simulink model "ConfiguredHevMmVirtualVehicle"  (R2025b)
settings: configuration reference "VehicleVariable" (kept outside this file)
StartFcn:
  | %tic
StopFcn:
  | %toc
model workspace (MAT data in the model file):
  ExtDrvCmdsSwitch : Simulink.Parameter (value not decoded)
  ExtDrvRefSwitch : Simulink.Parameter (value not decoded)
  ExtEnvSwitch : Simulink.Parameter (value not decoded)
  ExtGndSwitch : Simulink.Parameter (value not decoded)
symbols that are objects in the model workspace (value not decoded): ExtDrvCmdsSwitch, ExtDrvRefSwitch, ExtEnvSwitch, ExtGndSwitch
undefined symbols (not defined in the file or in its folder): AmbTemp, BaroPress, CurvGradRef, CurvRef, DCM, DriverAeroRes, DriverDrivelineRes, DriverInitialGear, DriverPreviewDist, DriverRollRes, DriverShiftTime, DriverTimeConst, DriverTractiveForce, EnvAbsPrs, EnvAirTemp, EnvGrvty, EnvNomFrictionScaling, EnvNominalGrade, EnvScnFrictionMap, EnvScnFrictionMapXBpts, EnvScnFrictionMapYBpts, EnvScnHeightMap, EnvScnHeightMapXBpts, EnvScnHeightMapYBpts, EnvWindVelX, EnvWindVelY, EnvWindVelZ, Gnd, Grade, HazzardCmd, HighBeamCmd, lambda_mux, LeftSignalCmd, LngRef, LowBeamCmd, LtrRef, PhiRef, PlntVehDstCGFrntAxl, PlntVehDstCGRearAxl, PlntVehInitLatPos, PlntVehInitLongPos, PlntVehInitPitchAng, PlntVehInitRollAng, PlntVehInitVertPos, PlntVehInitYawAng, PlntVehMass, PlntVehTrckWdth, PlntVehYawMomentInertia, PlntWhlLdRadiusFrnt, PlntWhlLdRadiusRear, RightSignalCmd, ScnCRRadius, Sim3dSensor, Wind, XRef, YRef, Z
libraries: simulink x28, autolibutils x8, autolibsharedcommon x7, vehdynlibscenariocommon x7, vehdynlibviscommon x4, vehdynlibdriver x2, sim3dgroundtruthsensorlib x2, sim3dlib x2, autolibshared x2, sim3dautolib x2, sl3dlib x1, sharedtransform x1
(part 5 of 6)

== system ConfiguredHevMmVirtualVehicle/Driver Commands/Driver Commands/Longitudinal Driver/Hill Hold & Stop ==
  LngRef : Inport
  <EnblDecelCmd> : Inport  Port=2
  <DecelOvrCmd> : Inport  Port=3
  <DecelHld> : Inport  Port=4
  <DecelZero> : Inport  Port=5
  Env : Inport  Port=6
  VehFdbk : Inport  Port=7
  Bus Selector : BusSelector  OutputSignals=Engine.EngSpdOut,Body.BdyFrm.Cg.Vel.xdot,Battery.BattInfo.BattSoc
  Bus Selector1 : BusSelector  OutputSignals=Body.BdyFrm.Cg.Vel.xdot
  Bus Selector2 : BusSelector  OutputSignals=Grade
  Hill Hold : Subsystem
  Logical Operator4 : Logic  Operator=OR  AllPortsSameDT=off  OutDataTypeStr=boolean
  Max : MinMax  Function=max  Inputs=2  ZeroCross=off
  Stop Detection : Subsystem
  Switch : Switch  Criteria=u2 > Threshold  SaturateOnIntegerOverflow=off  InputSameDT=off
  Switch1 : Switch  Criteria=u2 > Threshold  SaturateOnIntegerOverflow=off  InputSameDT=off
  VehFdbk1 : InportShadow  Port=7
  EnblDecelOvr : Outport
  DecelOvrCmd : Outport  Port=2
  DecelHld : Outport  Port=3
  DecelZero : Outport  Port=4
  VelFdbk : Outport  Port=5
  Grade : Outport  Port=6
  wires:
  Hill Hold/1(DecelOvr) -> Logical Operator4/1
  Hill Hold/2(EnblDecelOvr) -> Max/1
  Bus Selector/3 -> Hill Hold/3(<BattSoc>)  "<BattSoc>"
  Bus Selector/2 -> Hill Hold/2(<xdot>)  "<xdot>"
  Bus Selector/1 -> Hill Hold/1(<EngSpdOut>)  "<EngSpdOut>"
  Stop Detection/1(DecelOvrCmd) -> Max/2
  Stop Detection/2(EnblDecelOvr) -> Logical Operator4/2
  Logical Operator4/1 -> Switch/3
  Switch1/1 -> DecelOvrCmd/1
  Switch/1 -> EnblDecelOvr/1
  <EnblDecelCmd>/1 -> Switch1/2, Switch/1, Switch/2
  Max/1 -> Switch1/3
  Bus Selector1/1 -> VelFdbk/1, Stop Detection/2(<xdot>)  "<xdot>"
  LngRef/1 -> Hill Hold/4(LngRef), Stop Detection/1(LngRef)
  VehFdbk/1 -> Bus Selector/1
  <DecelOvrCmd>/1 -> Switch1/1
  Env/1 -> Bus Selector2/1
  Bus Selector2/1 -> Hill Hold/5(<Grade>), Grade/1  "<Grade>"
  VehFdbk1/1 -> Bus Selector1/1
  <DecelZero>/1 -> DecelZero/1
  <DecelHld>/1 -> DecelHld/1

== system ConfiguredHevMmVirtualVehicle/Driver Commands/Driver Commands/Longitudinal Driver/Longitudinal Driver ==
  VelRef : Inport  Unit=m/s
  EnblAccelOvr : Inport  Port=2
  AccelOvrCmd : Inport  Port=3
  AccelHld : Inport  Port=4
  AccelZero : Inport  Port=5
  EnblDecelOvr : Inport  Port=6
  DecelOvrCmd : Inport  Port=7
  DecelHld : Inport  Port=8
  DecelZero : Inport  Port=9
  VelFdbk : Inport  Port=10  Unit=m/s
  Grade : Inport  Port=11
  ExtGearGround : Ground
  External Action Routing : Subsystem
  Longitudinal Driver : autolibsharedcommon/Longitudinal Driver  cntrlType=PI  shftType=Reverse, Neutral, Drive  vnom=vnom  Kp=Kp  Ki=Ki  Kaw=Kaw  Kff=Kff  Kg=Kg  tauerr=tauerr  tShift=tShift  tRev=tRev  tPark=tPark  pdlVec=pdlVec  upShftTbl=upShftTbl  dwnShftTbl=dwnShftTbl  GearInit=GearInit  tClutch=tClutch  VehVelVec=VehVelVec  KffVec=KffVec  KiVec=KiVec  KpVec=KpVec  KgVec=KgVec  m=m  Kpt=Kpt  Lvv=L  g=g  UpGearVec=UpGearVec  DownGearVec=DownGearVec  aMode=6  errUnit=m/s  aR=aR  bR=bR  cR=cR  tauPt=tauPt
      settings: LibrarySourceBlock=autolibshared/Longitudinal Driver/Longitudinal Driver
  Info : Outport  InitialOutput=0  VectorParamsAs1DForOutWhenUnconnected=off
  AccelCmd : Outport  Port=2  VectorParamsAs1DForOutWhenUnconnected=off
  DecelCmd : Outport  Port=3  VectorParamsAs1DForOutWhenUnconnected=off
  GearCmd : Outport  Port=4
  wires:
  DecelZero/1 -> External Action Routing/8(DecelZero)
  DecelHld/1 -> External Action Routing/7(DecelHld)
  DecelOvrCmd/1 -> External Action Routing/6(DecelOvrCmd)
  EnblDecelOvr/1 -> External Action Routing/5(EnblDecelOvr)
  AccelZero/1 -> External Action Routing/4(AccelZero)
  AccelHld/1 -> External Action Routing/3(AccelHld)
  AccelOvrCmd/1 -> External Action Routing/2(AccelOvrCmd)
  EnblAccelOvr/1 -> External Action Routing/1(EnblAccelOvr)
  Longitudinal Driver/4 -> GearCmd/1
  ExtGearGround/1 -> Longitudinal Driver/4
  External Action Routing/1(ExtActions) -> Longitudinal Driver/5
  Grade/1 -> Longitudinal Driver/3
  Longitudinal Driver/3 -> DecelCmd/1
  Longitudinal Driver/2 -> AccelCmd/1
  Longitudinal Driver/1 -> Info/1
  VelFdbk/1 -> Longitudinal Driver/2
  VelRef/1 -> Longitudinal Driver/1

== system ConfiguredHevMmVirtualVehicle/Driver Commands/Driver Commands/Predictive Driver/Hill Hold & Stop ==
  LngRef : Inport
  <EnblDecelCmd> : Inport  Port=2
  <DecelOvrCmd> : Inport  Port=3
  <DecelHld> : Inport  Port=4
  <DecelZero> : Inport  Port=5
  Env : Inport  Port=6
  VehFdbk : Inport  Port=7
  Bus Selector : BusSelector  OutputSignals=Engine.EngSpdOut,Body.BdyFrm.Cg.Vel.xdot,Battery.BattInfo.BattSoc
  Bus Selector1 : BusSelector  OutputSignals=Body.BdyFrm.Cg.Vel.xdot
  Bus Selector2 : BusSelector  OutputSignals=Grade
  Hill Hold : Subsystem
  Logical Operator4 : Logic  Operator=OR  AllPortsSameDT=off  OutDataTypeStr=boolean
  Max : MinMax  Function=max  Inputs=2
  Stop Detection : Subsystem
  Switch : Switch  Criteria=u2 > Threshold  SaturateOnIntegerOverflow=off  InputSameDT=off
  Switch1 : Switch  Criteria=u2 > Threshold  SaturateOnIntegerOverflow=off  InputSameDT=off
  VehFdbk1 : InportShadow  Port=7
  EnblDecelOvr : Outport
  DecelOvrCmd : Outport  Port=2
  DecelHld : Outport  Port=3
  DecelZero : Outport  Port=4
  Grade : Outport  Port=5
  VelFdbk : Outport  Port=6
  wires:
  Hill Hold/1(DecelOvr) -> Logical Operator4/1
  Hill Hold/2(EnblDecelOvr) -> Max/1
  Bus Selector/3 -> Hill Hold/3(<BattSoc>)  "<BattSoc>"
  Bus Selector/2 -> Hill Hold/2(<xdot>)  "<xdot>"
  Bus Selector/1 -> Hill Hold/1(<EngSpdOut>)  "<EngSpdOut>"
  Stop Detection/1(DecelOvrCmd) -> Max/2
  Stop Detection/2(EnblDecelOvr) -> Logical Operator4/2
  Logical Operator4/1 -> Switch/3
  Switch1/1 -> DecelOvrCmd/1
  Switch/1 -> EnblDecelOvr/1
  <EnblDecelCmd>/1 -> Switch1/2, Switch/1, Switch/2
  Max/1 -> Switch1/3
  Bus Selector1/1 -> VelFdbk/1, Stop Detection/2(<xdot>)  "<xdot>"
  LngRef/1 -> Hill Hold/4(LngRef), Stop Detection/1(LngRef)
  VehFdbk/1 -> Bus Selector/1
  <DecelOvrCmd>/1 -> Switch1/1
  Env/1 -> Bus Selector2/1
  Bus Selector2/1 -> Hill Hold/5(<Grade>), Grade/1  "<Grade>"
  VehFdbk1/1 -> Bus Selector1/1
  <DecelZero>/1 -> DecelZero/1
  <DecelHld>/1 -> DecelHld/1

== system ConfiguredHevMmVirtualVehicle/Driver Commands/Driver Commands/Predictive Stanley Driver/Hill Hold & Stop ==
  LngRef : Inport
  <EnblDecelCmd> : Inport  Port=2
  <DecelOvrCmd> : Inport  Port=3
  <DecelHld> : Inport  Port=4
  <DecelZero> : Inport  Port=5
  <CurvRef> : Inport  Port=6
  Env : Inport  Port=7
  VehFdbk : Inport  Port=8
  Bus Selector : BusSelector  OutputSignals=Engine.EngSpdOut,Body.BdyFrm.Cg.Vel.xdot,Battery.BattInfo.BattSoc
  Bus Selector1 : BusSelector  OutputSignals=Body.BdyFrm.Cg.Vel.xdot
  Bus Selector2 : BusSelector  OutputSignals=Grade
  Hill Hold : Subsystem
  Logical Operator4 : Logic  Operator=OR  AllPortsSameDT=off  OutDataTypeStr=boolean
  Max : MinMax  Function=max  Inputs=2
  Stop Detection : Subsystem
  Switch : Switch  Criteria=u2 > Threshold  SaturateOnIntegerOverflow=off  InputSameDT=off
  Switch1 : Switch  Criteria=u2 > Threshold  SaturateOnIntegerOverflow=off  InputSameDT=off
  VehFdbk1 : InportShadow  Port=8
  EnblDecelOvr : Outport
  DecelOvrCmd : Outport  Port=2
  DecelHld : Outport  Port=3
  DecelZero : Outport  Port=4
  Grade : Outport  Port=5
  CurvRef : Outport  Port=6
  VelFdbk : Outport  Port=7
  wires:
  Hill Hold/1(DecelOvr) -> Logical Operator4/1
  Hill Hold/2(EnblDecelOvr) -> Max/1
  Bus Selector/3 -> Hill Hold/3(<BattSoc>)  "<BattSoc>"
  Bus Selector/2 -> Hill Hold/2(<xdot>)  "<xdot>"
  Bus Selector/1 -> Hill Hold/1(<EngSpdOut>)  "<EngSpdOut>"
  Stop Detection/1(DecelOvrCmd) -> Max/2
  Stop Detection/2(EnblDecelOvr) -> Logical Operator4/2
  Logical Operator4/1 -> Switch/3
  Switch1/1 -> DecelOvrCmd/1
  Switch/1 -> EnblDecelOvr/1
  <EnblDecelCmd>/1 -> Switch1/2, Switch/1, Switch/2
  Max/1 -> Switch1/3
  Bus Selector1/1 -> VelFdbk/1, Stop Detection/2(<xdot>)  "<xdot>"
  LngRef/1 -> Hill Hold/4(LngRef), Stop Detection/1(LngRef)
  <CurvRef>/1 -> CurvRef/1
  VehFdbk/1 -> Bus Selector/1
  <DecelOvrCmd>/1 -> Switch1/1
  Env/1 -> Bus Selector2/1
  Bus Selector2/1 -> Hill Hold/5(<Grade>), Grade/1  "<Grade>"
  VehFdbk1/1 -> Bus Selector1/1
  <DecelZero>/1 -> DecelZero/1
  <DecelHld>/1 -> DecelHld/1

== system ConfiguredHevMmVirtualVehicle/Environment/Ground Feedback/3D Engine/3D Engine Source ==
  WheelFdbk : Inport
  Multiple Points : Subsystem  VariantControl=terrType==2
  Single Point : Subsystem  VariantControl=terrType ==1
  z : Outport
  DCM : Outport  Port=2

== system ConfiguredHevMmVirtualVehicle/Environment/Ground Feedback/Height Map/2D Lookup Tbl for Elevation, Z ==
  XWhl : Inport  Partition=on  PartitionDimension=1  PartitionWidth=1  PartitionOffset=0
  YWhl : Inport  Port=2  Partition=on  PartitionDimension=1  PartitionWidth=1  PartitionOffset=0
  2-D Lookup Table : Lookup_n-D  BreakpointsForDimension1=EnvScnHeightMapXBpts  BreakpointsForDimension2=EnvScnHeightMapYBpts  BeginIndexSearchUsingPreviousIndexResult=on  Table=EnvScnHeightMap  ExtrapMethod=Clip  InternalRulePriority=Speed  RndMeth=Simplest
      settings: InputPortMap=u0,u1
  Add : Sum
  Add1 : Sum
  Constant : Constant  Value=0
  Constant1 : Constant  Value=0
  For Each : ForEach  DisableCoverage=on
  Unary Minus : UnaryMinus
  Z : Outport  ConcatenationDimension=1
  wires:
  2-D Lookup Table/1 -> Z/1
  YWhl/1 -> Unary Minus/1
  XWhl/1 -> Add1/2
  Unary Minus/1 -> Add/1
  Add/1 -> 2-D Lookup Table/2
  Constant/1 -> Add/2
  Constant1/1 -> Add1/1
  Add1/1 -> 2-D Lookup Table/1

== system ConfiguredHevMmVirtualVehicle/Environment/Ground Feedback/Height Map/Wheel Coordinates ==
  FrntAxlLftX : Inport
  FrntAxlRghtX : Inport  Port=2
  RearAxlLftX : Inport  Port=3
  RearAxlRghtX : Inport  Port=4
  FrntAxlLftY : Inport  Port=5
  FrntAxlRghtY : Inport  Port=6
  RearAxlLftY : Inport  Port=7
  RearAxlRghtY : Inport  Port=8
  Matrix Concatenate : Concatenate  NumInputs=4  Mode=Multidimensional array
  Matrix Concatenate1 : Concatenate  NumInputs=4  Mode=Multidimensional array
  XWhl : Outport
  YWhl : Outport  Port=2
  wires:
  Matrix Concatenate1/1 -> YWhl/1
  FrntAxlLftX/1 -> Matrix Concatenate/1
  FrntAxlLftY/1 -> Matrix Concatenate1/1
  FrntAxlRghtY/1 -> Matrix Concatenate1/2
  FrntAxlRghtX/1 -> Matrix Concatenate/2
  RearAxlLftY/1 -> Matrix Concatenate1/3
  RearAxlLftX/1 -> Matrix Concatenate/3
  RearAxlRghtY/1 -> Matrix Concatenate1/4
  Matrix Concatenate/1 -> XWhl/1
  RearAxlRghtX/1 -> Matrix Concatenate/4

== system ConfiguredHevMmVirtualVehicle/Environment/Ground Feedback/Ideal Inclined Plane/Ideal Inclined Plane ==
  X : Inport
  Y : Inport  Port=2
  phi : Inport  Port=3
  theta : Inport  Port=4
  Constant : Constant  Value=Z_est
  Enabled : Subsystem  Variant=on
  Signal Specification1 : SignalSpecification  Unit=rad
  Signal Specification3 : SignalSpecification  Unit=rad
  Signal Specification4 : SignalSpecification  Unit=m
  Signal Specification5 : SignalSpecification  Unit=m
  Signal Specification6 : SignalSpecification  Unit=m
  Z Plane : MATLAB Function  InitFcn=|  TreatAsAtomicUnit=on
      | if builtin('license','test','Vehicle_Dynamics_Blockset')
      |    [~]=builtin('license','checkout','Vehicle_Dynamics_Blockset');
      | else
      |    error(message('autoblks_shared:autosharederrAutoIcon:invalidLicense'));
      | end
      mask init:
      | if builtin('license','test','Vehicle_Dynamics_Blockset')
      |     [~]=builtin('license','checkout','Vehicle_Dynamics_Blockset');
      | else
      |     error(message('autoblks_shared:autosharederrAutoIcon:invalidLicense'));
      | end
  Z : Outport
  DCM : Outport  Port=2
  wires:
  Z Plane/2(DCM) -> DCM/1
  Signal Specification1/1 -> Z Plane/5(theta), Enabled/3(theta)
  phi/1 -> Signal Specification3/1
  theta/1 -> Signal Specification1/1
  Signal Specification3/1 -> Z Plane/4(phi), Enabled/2(phi)
  Y/1 -> Signal Specification6/1
  Z Plane/1(Z) -> Signal Specification4/1
  X/1 -> Signal Specification5/1
  Signal Specification4/1 -> Z/1
  Signal Specification5/1 -> Z Plane/1(X)
  Signal Specification6/1 -> Z Plane/2(Y)
  Constant/1 -> Enabled/1(Z), Z Plane/3(Zoffset)

== system ConfiguredHevMmVirtualVehicle/Environment/Ground Feedback/Ideal Inclined Plane/Wheel Coordinates ==
  FrntAxlLftX : Inport
  FrntAxlRghtX : Inport  Port=2
  RearAxlLftX : Inport  Port=3
  RearAxlRghtX : Inport  Port=4
  FrntAxlLftY : Inport  Port=5
  FrntAxlRghtY : Inport  Port=6
  RearAxlLftY : Inport  Port=7
  RearAxlRghtY : Inport  Port=8
  Matrix Concatenate : Concatenate  NumInputs=4  Mode=Multidimensional array
  Matrix Concatenate1 : Concatenate  NumInputs=4  Mode=Multidimensional array
  XWhl : Outport
  YWhl : Outport  Port=2
  wires:
  RearAxlRghtX/1 -> Matrix Concatenate/4
  Matrix Concatenate/1 -> XWhl/1
  RearAxlRghtY/1 -> Matrix Concatenate1/4
  RearAxlLftX/1 -> Matrix Concatenate/3
  RearAxlLftY/1 -> Matrix Concatenate1/3
  FrntAxlRghtX/1 -> Matrix Concatenate/2
  FrntAxlRghtY/1 -> Matrix Concatenate1/2
  FrntAxlLftY/1 -> Matrix Concatenate1/1
  FrntAxlLftX/1 -> Matrix Concatenate/1
  Matrix Concatenate1/1 -> YWhl/1

== system ConfiguredHevMmVirtualVehicle/Environment/Subsystem/Estimated Grade/Variant Subsystem ==
  note: 1) Add Subsystem or Model blocks as valid variant choices.
      | 2) You cannot connect blocks at this level. At simulation, connectivity is automatically
      | determined, based on the active variant and port name matching.
  Gnd : Inport
  Three-Axle : Subsystem  VariantControl=ThreeAxle
  Two-Axle : Subsystem  VariantControl=TwoAxle
  F : Outport
  R : Outport  Port=2

== system ConfiguredHevMmVirtualVehicle/Environment/Subsystem/Variant Subsystem/Three-Axle ==
  InGnd : Inport
  Bus Selector1 : BusSelector  OutputSignals=z.G_FL_z,z.G_FR_z,z.G_ML_z,z.G_MR_z,z.G_RL_z,z.G_RR_z,DCM,mu.mu_FL,mu.mu_FR,mu.mu_ML,mu.mu_MR,mu.mu_RL,mu.mu_RR
  Mux : Mux  Inputs=6
  Mux1 : Mux  Inputs=6
  z : Outport
  <DCM> : Outport  Port=2
  lambda_mux : Outport  Port=3
  wires:
  Bus Selector1/12 -> Mux1/5  "<mu_RL>"
  Bus Selector1/7 -> <DCM>/1  "<DCM>"
  InGnd/1 -> Bus Selector1/1
  Bus Selector1/10 -> Mux1/3  "<mu_ML>"
  Bus Selector1/4 -> Mux/4  "<G_MR_z>"
  Bus Selector1/5 -> Mux/5  "<G_RL_z>"
  Bus Selector1/3 -> Mux/3  "<G_ML_z>"
  Bus Selector1/2 -> Mux/2  "<G_FR_z>"
  Bus Selector1/9 -> Mux1/2  "<mu_FR>"
  Bus Selector1/6 -> Mux/6  "<G_RR_z>"
  Mux/1 -> z/1
  Bus Selector1/11 -> Mux1/4  "<mu_MR>"
  Bus Selector1/1 -> Mux/1  "<G_FL_z>"
  Bus Selector1/13 -> Mux1/6  "<mu_RR>"
  Mux1/1 -> lambda_mux/1
  Bus Selector1/8 -> Mux1/1  "<mu_FL>"

== system ConfiguredHevMmVirtualVehicle/Environment/Subsystem/Variant Subsystem/Two-Axle ==
  InGnd : Inport
  Bus Selector1 : BusSelector  OutputSignals=z.G_FL_z,z.G_FR_z,z.G_RL_z,z.G_RR_z,DCM,mu.mu_FL,mu.mu_FR,mu.mu_RL,mu.mu_RR
  Mux : Mux
  Mux1 : Mux
  z : Outport
  <DCM> : Outport  Port=2
  lambda_mux : Outport  Port=3
  wires:
  Bus Selector1/9 -> Mux1/4  "<mu_RR>"
  InGnd/1 -> Bus Selector1/1
  Bus Selector1/8 -> Mux1/3  "<mu_RL>"
  Bus Selector1/1 -> Mux/1  "<G_FL_z>"
  Bus Selector1/3 -> Mux/3  "<G_RL_z>"
  Bus Selector1/7 -> Mux1/2  "<mu_FR>"
  Bus Selector1/2 -> Mux/2  "<G_FR_z>"
  Bus Selector1/6 -> Mux1/1  "<mu_FL>"
  Bus Selector1/4 -> Mux/4  "<G_RR_z>"
  Mux1/1 -> lambda_mux/1
  Mux/1 -> z/1
  Bus Selector1/5 -> <DCM>/1  "<DCM>"

== system ConfiguredHevMmVirtualVehicle/Environment/Varying Friction/Friction Map/2D Lookup Tbl for Scaling Fctr (Lambda) ==
  XWhl : Inport  Partition=on  PartitionDimension=1  PartitionWidth=1  PartitionOffset=0
  YWhl : Inport  Port=2  Partition=on  PartitionDimension=1  PartitionWidth=1  PartitionOffset=0
  2-D Lookup Table : Lookup_n-D  BreakpointsForDimension1=EnvScnFrictionMapXBpts  BreakpointsForDimension2=EnvScnFrictionMapYBpts  BeginIndexSearchUsingPreviousIndexResult=on  Table=EnvScnFrictionMap  InterpMethod=Nearest  ExtrapMethod=Clip  InternalRulePriority=Speed  RndMeth=Simplest
      settings: InputPortMap=u0,u1
  Add : Sum
  Add1 : Sum
  Constant : Constant  Value=0
  Constant1 : Constant  Value=0
  For Each : ForEach  DisableCoverage=on
  Unary Minus : UnaryMinus
  FricCoeffLambda : Outport  ConcatenationDimension=1
  wires:
  2-D Lookup Table/1 -> FricCoeffLambda/1
  YWhl/1 -> Unary Minus/1
  Constant1/1 -> Add1/1
  Constant/1 -> Add/2
  Add/1 -> 2-D Lookup Table/2
  Add1/1 -> 2-D Lookup Table/1
  Unary Minus/1 -> Add/1
  XWhl/1 -> Add1/2

== system ConfiguredHevMmVirtualVehicle/Environment/Varying Friction/Friction Map/Wheel Coordinates ==
  FrntAxlLftX : Inport
  FrntAxlRghtX : Inport  Port=2
  RearAxlLftX : Inport  Port=3
  RearAxlRghtX : Inport  Port=4
  FrntAxlLftY : Inport  Port=5
  FrntAxlRghtY : Inport  Port=6
  RearAxlLftY : Inport  Port=7
  RearAxlRghtY : Inport  Port=8
  Matrix Concatenate : Concatenate  NumInputs=4  Mode=Multidimensional array
  Matrix Concatenate1 : Concatenate  NumInputs=4  Mode=Multidimensional array
  XWhl : Outport
  YWhl : Outport  Port=2
  wires:
  Matrix Concatenate1/1 -> YWhl/1
  FrntAxlLftX/1 -> Matrix Concatenate/1
  FrntAxlLftY/1 -> Matrix Concatenate1/1
  FrntAxlRghtY/1 -> Matrix Concatenate1/2
  FrntAxlRghtX/1 -> Matrix Concatenate/2
  RearAxlLftY/1 -> Matrix Concatenate1/3
  RearAxlLftX/1 -> Matrix Concatenate/3
  RearAxlRghtY/1 -> Matrix Concatenate1/4
  Matrix Concatenate/1 -> XWhl/1
  RearAxlRghtX/1 -> Matrix Concatenate/4

== system ConfiguredHevMmVirtualVehicle/Environment/Varying Friction/Varying Friction/Road Track Friction ==
  XWhl : Inport
  YWhl : Inport  Port=2
  Cg : Inport  Port=3
  2D Lookup Tbl for Scaling Fctr (Lambda) : Subsystem  TreatAsAtomicUnit=on
      mask init:
      | [~]=vehdynicon('vehdynblk',gcb);
  Bus Selector : BusSelector  OutputSignals=X,Y
  Cnst Lambda : Constant  Value=ones(4,1).*lambda_g
  Constant1 : Constant  Value=SplitLambdaTrck
  Creating Inertial Frm Bpt : Subsystem
  En at t = 0 : Subsystem
  "Lambda (t = 0) " : Memory  InitialCondition=ones(4,1).*lambda_g  InheritSampleTime=on
  Switch : Switch  Criteria=u2 > Threshold  SaturateOnIntegerOverflow=off  InputSameDT=off
  FricCoeffLambda : Outport
  wires:
  YWhl/1 -> 2D Lookup Tbl for Scaling Fctr (Lambda)/2(YWhl)
  XWhl/1 -> 2D Lookup Tbl for Scaling Fctr (Lambda)/1(XWhl)
  2D Lookup Tbl for Scaling Fctr (Lambda)/1(Lambda for each whl) -> Switch/1
  "Lambda (t = 0) "/1 -> FricCoeffLambda/1
  Switch/1 -> "Lambda (t = 0) "/1
  Cnst Lambda/1 -> Switch/3
  Constant1/1 -> Switch/2
  Cg/1 -> Bus Selector/1
  Creating Inertial Frm Bpt/1(XBpt) -> 2D Lookup Tbl for Scaling Fctr (Lambda)/3(XBpt)
  Creating Inertial Frm Bpt/2(YBpt) -> 2D Lookup Tbl for Scaling Fctr (Lambda)/4(YBpt)
  Bus Selector/1 -> Creating Inertial Frm Bpt/1(XCg)  "<X>"
  Bus Selector/2 -> Creating Inertial Frm Bpt/2(YCg)  "<Y>"
  En at t = 0/1(Out1) -> Creating Inertial Frm Bpt/Enable

== system ConfiguredHevMmVirtualVehicle/Environment/Varying Friction/Varying Friction/Wheel Coordinates ==
  FrntAxlLftX : Inport
  FrntAxlRghtX : Inport  Port=2
  RearAxlLftX : Inport  Port=3
  RearAxlRghtX : Inport  Port=4
  FrntAxlLftY : Inport  Port=5
  FrntAxlRghtY : Inport  Port=6
  RearAxlLftY : Inport  Port=7
  RearAxlRghtY : Inport  Port=8
  Matrix Concatenate : Concatenate  NumInputs=4  Mode=Multidimensional array
  Matrix Concatenate1 : Concatenate  NumInputs=4  Mode=Multidimensional array
  XWhl : Outport
  YWhl : Outport  Port=2
  wires:
  RearAxlRghtX/1 -> Matrix Concatenate/4
  Matrix Concatenate/1 -> XWhl/1
  RearAxlRghtY/1 -> Matrix Concatenate1/4
  RearAxlLftX/1 -> Matrix Concatenate/3
  RearAxlLftY/1 -> Matrix Concatenate1/3
  FrntAxlRghtX/1 -> Matrix Concatenate/2
  FrntAxlRghtY/1 -> Matrix Concatenate1/2
  FrntAxlLftY/1 -> Matrix Concatenate1/1
  FrntAxlLftX/1 -> Matrix Concatenate/1
  Matrix Concatenate1/1 -> YWhl/1

== system ConfiguredHevMmVirtualVehicle/Visualization/3D Engine/3D Engine/Part Rotation Concatenation ==
  Body Roll : Inport
  Body Ptich : Inport  Port=2
  Body Yaw : Inport  Port=3
  WheelFrontLeft Pitch : Inport  Port=4
  WheelFrontRight Pitch : Inport  Port=5
  WheelRearLeft Pitch : Inport  Port=6
  WheelRearRight Ptich : Inport  Port=7
  WheelFrontLeft Roll : Inport  Port=8
  WheelFrontRight Roll : Inport  Port=9
  WheelRearLeft Roll : Inport  Port=10
  WheelRearRight Roll : Inport  Port=11
  WheelFrontLeft Yaw : Inport  Port=12
  WheelFrontRight Yaw : Inport  Port=13
  WheelRearLeft Yaw : Inport  Port=14
  WheelRearRight Yaw : Inport  Port=15
  AllParts : Concatenate  NumInputs=5  Mode=Multidimensional array
  Body : Concatenate  NumInputs=3  Mode=Multidimensional array  ConcatenateDimension=2
  WheelFrontLeft : Concatenate  NumInputs=3  Mode=Multidimensional array  ConcatenateDimension=2
  WheelFrontRight : Concatenate  NumInputs=3  Mode=Multidimensional array  ConcatenateDimension=2
  WheelRearLeft : Concatenate  NumInputs=3  Mode=Multidimensional array  ConcatenateDimension=2
  WheelRearRight : Concatenate  NumInputs=3  Mode=Multidimensional array  ConcatenateDimension=2
  ConcatOut : Outport  VectorParamsAs1DForOutWhenUnconnected=off
  wires:
  WheelRearRight Roll/1 -> WheelRearRight/1
  WheelRearRight Ptich/1 -> WheelRearRight/2
  WheelRearLeft Roll/1 -> WheelRearLeft/1
  WheelRearLeft Pitch/1 -> WheelRearLeft/2
  WheelFrontRight Roll/1 -> WheelFrontRight/1
  WheelFrontRight Pitch/1 -> WheelFrontRight/2
  WheelFrontLeft Roll/1 -> WheelFrontLeft/1
  WheelFrontLeft Pitch/1 -> WheelFrontLeft/2
  Body Roll/1 -> Body/1
  Body Ptich/1 -> Body/2
  WheelFrontRight Yaw/1 -> WheelFrontRight/3
  WheelRearRight/1 -> AllParts/5
  AllParts/1 -> ConcatOut/1
  WheelRearLeft Yaw/1 -> WheelRearLeft/3
  WheelRearRight Yaw/1 -> WheelRearRight/3
  WheelFrontRight/1 -> AllParts/3
  WheelRearLeft/1 -> AllParts/4
  Body/1 -> AllParts/1
  WheelFrontLeft/1 -> AllParts/2
  WheelFrontLeft Yaw/1 -> WheelFrontLeft/3
  Body Yaw/1 -> Body/3

== system ConfiguredHevMmVirtualVehicle/Visualization/3D Engine/3D Engine/Part Translation Concatenation ==
  BodyX : Inport
  BodyY : Inport  Port=2
  BodyZ : Inport  Port=3
  WheelFrontLeftX : Inport  Port=4
  WheelFrontRightX : Inport  Port=5
  WheelRearLeftX : Inport  Port=6
  WheelRearRightX : Inport  Port=7
  WheelFrontLeftY : Inport  Port=8
  WheelFrontRightY : Inport  Port=9
  WheelRearLeftY : Inport  Port=10
  WheelRearRightY : Inport  Port=11
  WheelFrontLeftZ : Inport  Port=12
  WheelFrontRightZ : Inport  Port=13
  WheelRearLeftZ : Inport  Port=14
  WheelRearRightZ : Inport  Port=15
  AllParts : Concatenate  NumInputs=5  Mode=Multidimensional array
  Body : Concatenate  NumInputs=3  Mode=Multidimensional array  ConcatenateDimension=2
  WheelFrontLeft : Concatenate  NumInputs=3  Mode=Multidimensional array  ConcatenateDimension=2
  WheelFrontRight : Concatenate  NumInputs=3  Mode=Multidimensional array  ConcatenateDimension=2
  WheelRearLeft : Concatenate  NumInputs=3  Mode=Multidimensional array  ConcatenateDimension=2
  WheelRearRight : Concatenate  NumInputs=3  Mode=Multidimensional array  ConcatenateDimension=2
  ConcatOut : Outport  VectorParamsAs1DForOutWhenUnconnected=off
  wires:
  WheelFrontRightZ/1 -> WheelFrontRight/3
  WheelRearLeftX/1 -> WheelRearLeft/1
  WheelRearRight/1 -> AllParts/5
  WheelRearLeftY/1 -> WheelRearLeft/2
  AllParts/1 -> ConcatOut/1
  WheelRearLeftZ/1 -> WheelRearLeft/3
  WheelRearRightY/1 -> WheelRearRight/2
  WheelFrontRightX/1 -> WheelFrontRight/1
  WheelFrontRightY/1 -> WheelFrontRight/2
  WheelRearRightZ/1 -> WheelRearRight/3
  WheelFrontRight/1 -> AllParts/3
  WheelRearLeft/1 -> AllParts/4
  Body/1 -> AllParts/1
  WheelRearRightX/1 -> WheelRearRight/1
  WheelFrontLeft/1 -> AllParts/2
  BodyY/1 -> Body/2
  WheelFrontLeftY/1 -> WheelFrontLeft/2
  WheelFrontLeftZ/1 -> WheelFrontLeft/3
  WheelFrontLeftX/1 -> WheelFrontLeft/1
  BodyZ/1 -> Body/3
  BodyX/1 -> Body/1

== system ConfiguredHevMmVirtualVehicle/Visualization/3D Engine/3D Engine/Scale ==
  Constant{1..12,17,32..33} (15 alike) : Constant  OutDataTypeStr=single
  PartConcatenation : Subsystem
  ScaleOut : Outport  VectorParamsAs1DForOutWhenUnconnected=off
  wires:
  PartConcatenation/1(ConcatOut) -> ScaleOut/1
  Constant12/1 -> PartConcatenation/1(BodyX)
  Constant17/1 -> PartConcatenation/2(BodyY)
  Constant32/1 -> PartConcatenation/3(BodyZ)
  Constant33/1 -> PartConcatenation/4(WheelFrontLeftX)
  Constant1/1 -> PartConcatenation/5(WheelFrontLeftY)
  Constant2/1 -> PartConcatenation/6(WheelFrontLeftZ)
  Constant5/1 -> PartConcatenation/7(WheelFrontRightX)
  Constant3/1 -> PartConcatenation/8(WheelFrontRightY)
  Constant4/1 -> PartConcatenation/9(WheelFrontRightZ)
  Constant8/1 -> PartConcatenation/10(WheelRearLeftX)
  Constant6/1 -> PartConcatenation/11(WheelRearLeftY)
  Constant7/1 -> PartConcatenation/12(WheelRearLeftZ)
  Constant11/1 -> PartConcatenation/13(WheelRearRightX)
  Constant9/1 -> PartConcatenation/14(WheelRearRightY)
  Constant10/1 -> PartConcatenation/15(WheelRearRightZ)

== system ConfiguredHevMmVirtualVehicle/Visualization/3D Engine/3D Engine/Trailer ==
  note: 1) Add Subsystem or Model blocks as valid variant choices.
      | 2) You cannot connect blocks at this level. At simulation, connectivity is automatically
      | determined, based on the active variant and port name matching.
  VehFdbk : Inport
  No Trailer : Subsystem  VariantControl=No Trailer
  One-Axle Trailer : Subsystem  VariantControl=One-Axle Trailer

== system ConfiguredHevMmVirtualVehicle/Visualization/Vehicle XY Plotter/XY View/Driveline Speed ==
  <EngSpd> : Inport
  <EMSpd> : Inport  Port=2
  Abs : Abs  ZeroCross=off  SaturateOnIntegerOverflow=off
  Abs1 : Abs  ZeroCross=off  SaturateOnIntegerOverflow=off
  Divide : Product  Inputs=*/
  Probe Dimension : Probe  ProbeWidth=off  ProbeSampleTime=off  ProbeComplexSignal=off  ProbeSignalDimensions=on
  Relational Operator : RelationalOperator  Operator=<=  OutDataTypeStr=boolean  ZeroCross=off  RndMeth=Simplest  InputSameDT=off
  Sum of Elements : Sum  Inputs=+
  Switch : Switch  Criteria=u2 > Threshold  ZeroCross=off  SaturateOnIntegerOverflow=off  InputSameDT=off
  MaxSpd : Outport
  wires:
  Switch/1 -> MaxSpd/1
  Sum of Elements/1 -> Divide/1
  Probe Dimension/1 -> Divide/2
  Divide/1 -> Switch/3, Abs1/1
  <EngSpd>/1 -> Switch/1, Abs/1
  Abs/1 -> Relational Operator/2
  <EMSpd>/1 -> Probe Dimension/1, Sum of Elements/1
  Relational Operator/1 -> Switch/2
  Abs1/1 -> Relational Operator/1

== system ConfiguredHevMmVirtualVehicle/Visualization/Vehicle XY Plotter/XY View Ref/Driveline Speed ==
  <EngSpd> : Inport
  <EMSpd> : Inport  Port=2
  Abs : Abs  ZeroCross=off  SaturateOnIntegerOverflow=off
  Abs1 : Abs  ZeroCross=off  SaturateOnIntegerOverflow=off
  Divide : Product  Inputs=*/
  Probe Dimension : Probe  ProbeWidth=off  ProbeSampleTime=off  ProbeComplexSignal=off  ProbeSignalDimensions=on
  Relational Operator : RelationalOperator  Operator=<=  OutDataTypeStr=boolean  ZeroCross=off  RndMeth=Simplest  InputSameDT=off
  Sum of Elements : Sum  Inputs=+
  Switch : Switch  Criteria=u2 > Threshold  ZeroCross=off  SaturateOnIntegerOverflow=off  InputSameDT=off
  MaxSpd : Outport
  wires:
  Switch/1 -> MaxSpd/1
  Sum of Elements/1 -> Divide/1
  Probe Dimension/1 -> Divide/2
  Divide/1 -> Switch/3, Abs1/1
  <EngSpd>/1 -> Switch/1, Abs/1
  Abs/1 -> Relational Operator/2
  <EMSpd>/1 -> Probe Dimension/1, Sum of Elements/1
  Relational Operator/1 -> Switch/2
  Abs1/1 -> Relational Operator/1

== system ConfiguredHevMmVirtualVehicle/Visualization/Vehicle XY Plotter/XY View Ref with One-Axle Trailer/Driveline Speed ==
  <EngSpd> : Inport
  <EMSpd> : Inport  Port=2
  Abs : Abs  ZeroCross=off  SaturateOnIntegerOverflow=off
  Abs1 : Abs  ZeroCross=off  SaturateOnIntegerOverflow=off
  Divide : Product  Inputs=*/
  Probe Dimension : Probe  ProbeWidth=off  ProbeSampleTime=off  ProbeComplexSignal=off  ProbeSignalDimensions=on
  Relational Operator : RelationalOperator  Operator=<=  OutDataTypeStr=boolean  ZeroCross=off  RndMeth=Simplest  InputSameDT=off
  Sum of Elements : Sum  Inputs=+
  Switch : Switch  Criteria=u2 > Threshold  ZeroCross=off  SaturateOnIntegerOverflow=off  InputSameDT=off
  MaxSpd : Outport
  wires:
  Switch/1 -> MaxSpd/1
  Sum of Elements/1 -> Divide/1
  Probe Dimension/1 -> Divide/2
  Divide/1 -> Switch/3, Abs1/1
  <EngSpd>/1 -> Switch/1, Abs/1
  Abs/1 -> Relational Operator/2
  <EMSpd>/1 -> Probe Dimension/1, Sum of Elements/1
  Relational Operator/1 -> Switch/2
  Abs1/1 -> Relational Operator/1

== system ConfiguredHevMmVirtualVehicle/Driver Commands/Driver Commands/Longitudinal Driver/Hill Hold & Stop/Hill Hold ==
  <EngSpdOut> : Inport
  <xdot> : Inport  Port=2
  <BattSoc> : Inport  Port=3
  LngRef : Inport  Port=4
  <Grade> : Inport  Port=5
  Abs : Abs  ZeroCross=off  SaturateOnIntegerOverflow=off
  Abs1 : Abs  ZeroCross=off  SaturateOnIntegerOverflow=off
  Compare To Constant : simulink/Logic and Bit Operations/Compare To Constant  relop=<=  const=.1  OutDataTypeStr=boolean  ZeroCross=off
  Compare To Constant1 : simulink/Logic and Bit Operations/Compare To Constant  relop=>=  const=.1  OutDataTypeStr=boolean  ZeroCross=off
  Compare To Constant2 : simulink/Logic and Bit Operations/Compare To Constant  relop=<=  const=500  OutDataTypeStr=boolean  ZeroCross=off
  Compare To Constant3 : simulink/Logic and Bit Operations/Compare To Constant  relop=<=  const=5  OutDataTypeStr=boolean  ZeroCross=off
  Compare To Constant4 : simulink/Logic and Bit Operations/Compare To Constant  relop=<=  const=.1  OutDataTypeStr=boolean  ZeroCross=off
  Data Type Conversion1 : DataTypeConversion  SaturateOnIntegerOverflow=off  RndMeth=Floor
  Logical Operator : Logic  AllPortsSameDT=off  OutDataTypeStr=boolean
  Logical Operator1 : Logic  Inputs=3  AllPortsSameDT=off  OutDataTypeStr=boolean
  Logical Operator2 : Logic  Operator=OR  AllPortsSameDT=off  OutDataTypeStr=boolean
  Signal Specification : SignalSpecification  Unit=m/s
  Unit Conversion : UnitConversion
  DecelOvr : Outport
  EnblDecelOvr : Outport  Port=2
  wires:
  <BattSoc>/1 -> Compare To Constant4/1
  <xdot>/1 -> Unit Conversion/1
  <Grade>/1 -> Abs1/1
  Compare To Constant4/1 -> Logical Operator1/3
  <EngSpdOut>/1 -> Compare To Constant2/1
  Signal Specification/1 -> Compare To Constant3/1
  Abs/1 -> Compare To Constant/1
  Logical Operator1/1 -> Logical Operator2/1
  Data Type Conversion1/1 -> EnblDecelOvr/1
  Compare To Constant2/1 -> Logical Operator1/1
  Logical Operator/1 -> Logical Operator2/2
  Compare To Constant3/1 -> Logical Operator1/2
  Compare To Constant1/1 -> Logical Operator/2
  LngRef/1 -> Abs/1
  Abs1/1 -> Compare To Constant1/1
  Logical Operator2/1 -> Data Type Conversion1/1, DecelOvr/1
  Unit Conversion/1 -> Signal Specification/1
  Compare To Constant/1 -> Logical Operator/1

== system ConfiguredHevMmVirtualVehicle/Driver Commands/Driver Commands/Longitudinal Driver/Hill Hold & Stop/Stop Detection ==
  LngRef : Inport
  <xdot> : Inport  Port=2
  Abs2 : Abs  ZeroCross=off  SaturateOnIntegerOverflow=off
  Compare To Constant5 : simulink/Logic and Bit Operations/Compare To Constant  relop=<=  const=.1  OutDataTypeStr=boolean  ZeroCross=off
  Compare To Constant6 : simulink/Logic and Bit Operations/Compare To Constant  relop===  const=0  OutDataTypeStr=boolean  ZeroCross=off
  Cont LPF : autolibutils/Cont LPF  wc=2*pi*40  AbsoluteTolerance=auto  aMode=6
  Data Type Conversion2 : DataTypeConversion  SaturateOnIntegerOverflow=off  RndMeth=Floor
  Gain : Gain  Gain=.1
  LatchSwitchCont : autolibutils/LatchSwitchCont  aMode=6
  Logical Operator1 : Logic  Operator=NOT  AllPortsSameDT=off  OutDataTypeStr=boolean
  Logical Operator3 : Logic  AllPortsSameDT=off  OutDataTypeStr=boolean
  DecelOvrCmd : Outport
  EnblDecelOvr : Outport  Port=2
  wires:
  <xdot>/1 -> Abs2/1
  Cont LPF/1 -> DecelOvrCmd/1
  Gain/1 -> Cont LPF/1
  Compare To Constant6/1 -> Logical Operator3/2, Logical Operator1/1
  Logical Operator1/1 -> LatchSwitchCont/2
  Data Type Conversion2/1 -> Gain/1
  LatchSwitchCont/1 -> Data Type Conversion2/1, EnblDecelOvr/1
  Abs2/1 -> Compare To Constant5/1
  LngRef/1 -> Compare To Constant6/1
  Logical Operator3/1 -> LatchSwitchCont/1
  Compare To Constant5/1 -> Logical Operator3/1

== system ConfiguredHevMmVirtualVehicle/Driver Commands/Driver Commands/Longitudinal Driver/Longitudinal Driver/External Action Routing ==
  EnblAccelOvr : Inport  OutDataTypeStr=boolean  Unit=1  PortDimensions=1
  AccelOvrCmd : Inport  Port=2  OutDataTypeStr=double  Unit=1  PortDimensions=1
  AccelHld : Inport  Port=3  OutDataTypeStr=boolean  Unit=1  PortDimensions=1
  AccelZero : Inport  Port=4  OutDataTypeStr=boolean  Unit=1  PortDimensions=1
  EnblDecelOvr : Inport  Port=5  OutDataTypeStr=boolean  Unit=1  PortDimensions=1
  DecelOvrCmd : Inport  Port=6  OutDataTypeStr=double  Unit=1  PortDimensions=1
  DecelHld : Inport  Port=7  OutDataTypeStr=boolean  Unit=1  PortDimensions=1
  DecelZero : Inport  Port=8  OutDataTypeStr=boolean  Unit=1  PortDimensions=1
  Bus Creator2 : BusCreator  Inputs=8
  ExtActions : Outport
  wires:
  Bus Creator2/1 -> ExtActions/1  "ExtActions"
  DecelZero/1 -> Bus Creator2/8  "DecelZero"
  DecelHld/1 -> Bus Creator2/7  "DecelHld"
  DecelOvrCmd/1 -> Bus Creator2/6  "DecelOvrCmd"
  EnblDecelOvr/1 -> Bus Creator2/5  "EnblDecelOvr"
  AccelZero/1 -> Bus Creator2/4  "AccelZero"
  AccelHld/1 -> Bus Creator2/3  "AccelHld"
  AccelOvrCmd/1 -> Bus Creator2/2  "AccelOvrCmd"
  EnblAccelOvr/1 -> Bus Creator2/1  "EnblAccelOvr"

== system ConfiguredHevMmVirtualVehicle/Driver Commands/Driver Commands/Predictive Driver/Hill Hold & Stop/Hill Hold ==
  <EngSpdOut> : Inport
  <xdot> : Inport  Port=2
  <BattSoc> : Inport  Port=3
  LngRef : Inport  Port=4
  <Grade> : Inport  Port=5
  Abs : Abs  ZeroCross=off  SaturateOnIntegerOverflow=off
  Abs1 : Abs  ZeroCross=off  SaturateOnIntegerOverflow=off
  Compare To Constant : simulink/Logic and Bit Operations/Compare To Constant  relop=<=  const=.1  OutDataTypeStr=boolean  ZeroCross=off
  Compare To Constant1 : simulink/Logic and Bit Operations/Compare To Constant  relop=>=  const=.1  OutDataTypeStr=boolean  ZeroCross=off
  Compare To Constant2 : simulink/Logic and Bit Operations/Compare To Constant  relop=<=  const=500  OutDataTypeStr=boolean  ZeroCross=off
  Compare To Constant3 : simulink/Logic and Bit Operations/Compare To Constant  relop=<=  const=5  OutDataTypeStr=boolean  ZeroCross=off
  Compare To Constant4 : simulink/Logic and Bit Operations/Compare To Constant  relop=<=  const=.1  OutDataTypeStr=boolean  ZeroCross=off
  Data Type Conversion1 : DataTypeConversion  SaturateOnIntegerOverflow=off  RndMeth=Floor
  Logical Operator : Logic  AllPortsSameDT=off  OutDataTypeStr=boolean
  Logical Operator1 : Logic  Inputs=3  AllPortsSameDT=off  OutDataTypeStr=boolean
  Logical Operator2 : Logic  Operator=OR  AllPortsSameDT=off  OutDataTypeStr=boolean
  Signal Specification : SignalSpecification  Unit=m/s
  Unit Conversion : UnitConversion
  DecelOvr : Outport
  EnblDecelOvr : Outport  Port=2
  wires:
  <BattSoc>/1 -> Compare To Constant4/1
  <xdot>/1 -> Unit Conversion/1
  <Grade>/1 -> Abs1/1
  Compare To Constant4/1 -> Logical Operator1/3
  <EngSpdOut>/1 -> Compare To Constant2/1
  Signal Specification/1 -> Compare To Constant3/1
  Abs/1 -> Compare To Constant/1
  Logical Operator1/1 -> Logical Operator2/1
  Data Type Conversion1/1 -> EnblDecelOvr/1
  Compare To Constant2/1 -> Logical Operator1/1
  Logical Operator/1 -> Logical Operator2/2
  Compare To Constant3/1 -> Logical Operator1/2
  Compare To Constant1/1 -> Logical Operator/2
  LngRef/1 -> Abs/1
  Abs1/1 -> Compare To Constant1/1
  Logical Operator2/1 -> Data Type Conversion1/1, DecelOvr/1
  Unit Conversion/1 -> Signal Specification/1
  Compare To Constant/1 -> Logical Operator/1

== system ConfiguredHevMmVirtualVehicle/Driver Commands/Driver Commands/Predictive Driver/Hill Hold & Stop/Stop Detection ==
  LngRef : Inport
  <xdot> : Inport  Port=2
  Abs2 : Abs  ZeroCross=off  SaturateOnIntegerOverflow=off
  Compare To Constant5 : simulink/Logic and Bit Operations/Compare To Constant  relop=<=  const=.1  OutDataTypeStr=boolean  ZeroCross=off
  Compare To Constant6 : simulink/Logic and Bit Operations/Compare To Constant  relop===  const=0  OutDataTypeStr=boolean  ZeroCross=off
  Cont LPF : autolibutils/Cont LPF  wc=2*pi*40  AbsoluteTolerance=auto  aMode=6
  Data Type Conversion2 : DataTypeConversion  SaturateOnIntegerOverflow=off  RndMeth=Floor
  Gain : Gain  Gain=.1
  LatchSwitchCont : autolibutils/LatchSwitchCont  aMode=6
  Logical Operator1 : Logic  Operator=NOT  AllPortsSameDT=off  OutDataTypeStr=boolean
  Logical Operator3 : Logic  AllPortsSameDT=off  OutDataTypeStr=boolean
  DecelOvrCmd : Outport
  EnblDecelOvr : Outport  Port=2
  wires:
  <xdot>/1 -> Abs2/1
  Cont LPF/1 -> DecelOvrCmd/1
  Gain/1 -> Cont LPF/1
  Compare To Constant6/1 -> Logical Operator3/2, Logical Operator1/1
  Logical Operator1/1 -> LatchSwitchCont/2
  Data Type Conversion2/1 -> Gain/1
  LatchSwitchCont/1 -> Data Type Conversion2/1, EnblDecelOvr/1
  Abs2/1 -> Compare To Constant5/1
  LngRef/1 -> Compare To Constant6/1
  Logical Operator3/1 -> LatchSwitchCont/1
  Compare To Constant5/1 -> Logical Operator3/1

== system ConfiguredHevMmVirtualVehicle/Driver Commands/Driver Commands/Predictive Stanley Driver/Hill Hold & Stop/Hill Hold ==
  <EngSpdOut> : Inport
  <xdot> : Inport  Port=2
  <BattSoc> : Inport  Port=3
  LngRef : Inport  Port=4
  <Grade> : Inport  Port=5
  Abs : Abs  ZeroCross=off  SaturateOnIntegerOverflow=off
  Abs1 : Abs  ZeroCross=off  SaturateOnIntegerOverflow=off
  Compare To Constant : simulink/Logic and Bit Operations/Compare To Constant  relop=<=  const=.1  OutDataTypeStr=boolean  ZeroCross=off
  Compare To Constant1 : simulink/Logic and Bit Operations/Compare To Constant  relop=>=  const=.1  OutDataTypeStr=boolean  ZeroCross=off
  Compare To Constant2 : simulink/Logic and Bit Operations/Compare To Constant  relop=<=  const=500  OutDataTypeStr=boolean  ZeroCross=off
  Compare To Constant3 : simulink/Logic and Bit Operations/Compare To Constant  relop=<=  const=5  OutDataTypeStr=boolean  ZeroCross=off
  Compare To Constant4 : simulink/Logic and Bit Operations/Compare To Constant  relop=<=  const=.1  OutDataTypeStr=boolean  ZeroCross=off
  Data Type Conversion1 : DataTypeConversion  SaturateOnIntegerOverflow=off  RndMeth=Floor
  Logical Operator : Logic  AllPortsSameDT=off  OutDataTypeStr=boolean
  Logical Operator1 : Logic  Inputs=3  AllPortsSameDT=off  OutDataTypeStr=boolean
  Logical Operator2 : Logic  Operator=OR  AllPortsSameDT=off  OutDataTypeStr=boolean
  Signal Specification : SignalSpecification  Unit=m/s
  Unit Conversion : UnitConversion
  DecelOvr : Outport
  EnblDecelOvr : Outport  Port=2
  wires:
  <BattSoc>/1 -> Compare To Constant4/1
  <xdot>/1 -> Unit Conversion/1
  <Grade>/1 -> Abs1/1
  Compare To Constant4/1 -> Logical Operator1/3
  <EngSpdOut>/1 -> Compare To Constant2/1
  Signal Specification/1 -> Compare To Constant3/1
  Abs/1 -> Compare To Constant/1
  Logical Operator1/1 -> Logical Operator2/1
  Data Type Conversion1/1 -> EnblDecelOvr/1
  Compare To Constant2/1 -> Logical Operator1/1
  Logical Operator/1 -> Logical Operator2/2
  Compare To Constant3/1 -> Logical Operator1/2
  Compare To Constant1/1 -> Logical Operator/2
  LngRef/1 -> Abs/1
  Abs1/1 -> Compare To Constant1/1
  Logical Operator2/1 -> Data Type Conversion1/1, DecelOvr/1
  Unit Conversion/1 -> Signal Specification/1
  Compare To Constant/1 -> Logical Operator/1

== system ConfiguredHevMmVirtualVehicle/Driver Commands/Driver Commands/Predictive Stanley Driver/Hill Hold & Stop/Stop Detection ==
  LngRef : Inport
  <xdot> : Inport  Port=2
  Abs2 : Abs  ZeroCross=off  SaturateOnIntegerOverflow=off
  Compare To Constant5 : simulink/Logic and Bit Operations/Compare To Constant  relop=<=  const=.1  OutDataTypeStr=boolean  ZeroCross=off
  Compare To Constant6 : simulink/Logic and Bit Operations/Compare To Constant  relop===  const=0  OutDataTypeStr=boolean  ZeroCross=off
  Cont LPF : autolibutils/Cont LPF  wc=2*pi*40  AbsoluteTolerance=auto  aMode=6
  Data Type Conversion2 : DataTypeConversion  SaturateOnIntegerOverflow=off  RndMeth=Floor
  Gain : Gain  Gain=.1
  LatchSwitchCont : autolibutils/LatchSwitchCont  aMode=6
  Logical Operator1 : Logic  Operator=NOT  AllPortsSameDT=off  OutDataTypeStr=boolean
  Logical Operator3 : Logic  AllPortsSameDT=off  OutDataTypeStr=boolean
  DecelOvrCmd : Outport
  EnblDecelOvr : Outport  Port=2
  wires:
  <xdot>/1 -> Abs2/1
  Cont LPF/1 -> DecelOvrCmd/1
  Gain/1 -> Cont LPF/1
  Compare To Constant6/1 -> Logical Operator3/2, Logical Operator1/1
  Logical Operator1/1 -> LatchSwitchCont/2
  Data Type Conversion2/1 -> Gain/1
  LatchSwitchCont/1 -> Data Type Conversion2/1, EnblDecelOvr/1
  Abs2/1 -> Compare To Constant5/1
  LngRef/1 -> Compare To Constant6/1
  Logical Operator3/1 -> LatchSwitchCont/1
  Compare To Constant5/1 -> Logical Operator3/1
